simulink model "sschdlexVariableResistorModel"  (R2026a)
settings: Solver=VariableStepAuto  StopTime=.25
libraries: fl_lib x5, nesl_utility x4
settings Model: Creator=The MathWorks, Inc.  LastModifiedBy=The MathWorks, Inc.
settings SimscapeCC: SimscapeNominalValues="[{\"value\":\"1\",\"unit\":\"A\"},{\"value\":\"1\",\"unit\":\"bar\"},{\"value\":\"1\",\"unit\":\"cm^2\"},{\"value\":\"1\",\"unit\":\"cm^3/s\"},{\"value\":\"1\",\"unit\":\"kJ/kg\"},{\"value\":\"1\",\"unit\":\"kW\"},{\"value\":\"1\",\"unit\":\"l\"},{\"value\":\"1\",\"unit\":\"N\"},{\"value\":\"1\",\"unit\":\"N*m\"},{\"value\":\"1\",\"unit\":\"V\"}]"  SimscapeLogType=none  SimscapeLogDataHistory=5000.0

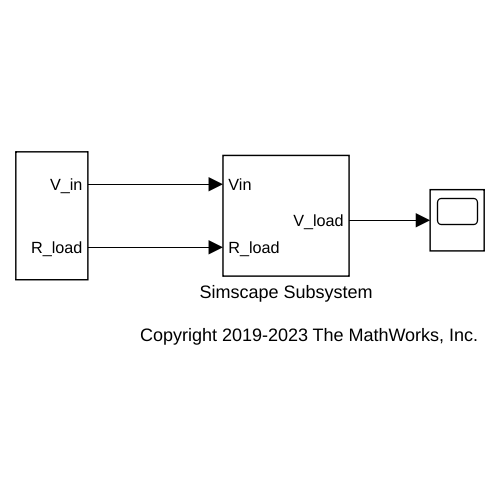
[thumbnail: Simulink's stored preview of the top-level diagram]
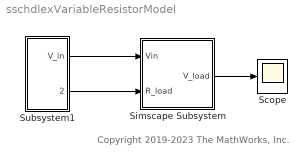
== system sschdlexVariableResistorModel ==
  note: Copyright 2019-2023 The MathWorks, Inc.
  Scope : Scope
      settings: ActiveDisplayYMinimum=-1.68736  ActiveDisplayYMaximum=15.18624
  Simscape Subsystem : Subsystem
  Subsystem1 : Subsystem
  wires:
  Simscape Subsystem/1(V_load) -> Scope/1
  Subsystem1/1(V_in) -> Simscape Subsystem/1(Vin)
  Subsystem1/2(R_load) -> Simscape Subsystem/2(R_load)

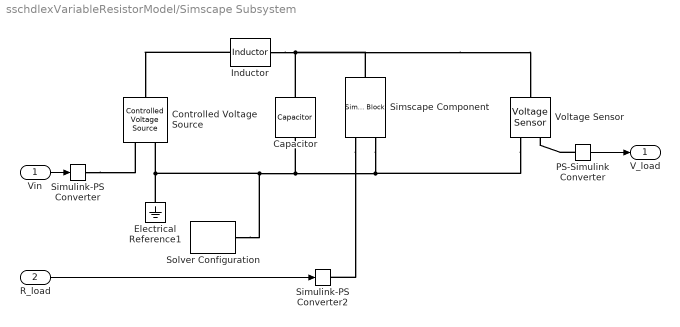
== system sschdlexVariableResistorModel/Simscape Subsystem ==
  Vin : Inport
  R_load : Inport  Port=2
  Capacitor : fl_lib/Electrical/Electrical Elements/Capacitor  c=1e-6 F  r=1e-6 Ohm  g=0 1/Ohm  i_specify=off  i_priority=None  i=0 A  i_nominal_specify=off  i_nominal_value=1  i_nominal_unit=A  v_specify=off  v_priority=None  v=0 V  v_nominal_specify=off  v_nominal_value=1  v_nominal_unit=V  vc_specify=off  vc_priority=High  vc=0 V  vc_nominal_specify=off  vc_nominal_value=1  vc_nominal_unit=V
  Controlled Voltage Source : fl_lib/Electrical/Electrical Sources/Controlled Voltage Source
  Electrical Reference1 : fl_lib/Electrical/Electrical Elements/Electrical Reference
  Inductor : fl_lib/Electrical/Electrical Elements/Inductor  l=1e-3 H  r=0 Ohm  g=1e-9 1/Ohm  i_specify=off  i_priority=None  i=0 A  i_nominal_specify=off  i_nominal_value=1  i_nominal_unit=A  v_specify=off  v_priority=None  v=0 V  v_nominal_specify=off  v_nominal_value=1  v_nominal_unit=V  i_L_specify=off  i_L_priority=High  i_L=0 A  i_L_nominal_specify=off  i_L_nominal_value=1  i_L_nominal_unit=A
  PS-Simulink Converter : nesl_utility/PS-Simulink Converter  PhysicalDomain=network_engine_domain  SubClassName=ps_output  LeftPortType=input  RightPortType=output  PseudoPeriodic=off  Frequencies=[]  VectorFormat=1-D array  Unit=1  AffineConversion=off
  Simscape Component : SimscapeComponentBlock  SourceFile=PiecewiseConstantResistor  ComponentPath=PiecewiseConstantResistor  ComponentVariants="[\"PiecewiseConstantResistor\"]"  ComponentVariantNames="[\"PiecewiseConstantResistor\"]"  ClassName=PiecewiseConstantResistor  SchemaVersion=1  Rmin=1e-6 Ohm  Rtol=1e-6 Ohm  i_specify=off  i_priority=None  i=0 A  i_nominal_specify=off  i_nominal_value=1  i_nominal_unit=A  v_specify=off  v_priority=None  v=0 V  v_nominal_specify=off  v_nominal_value=1  v_nominal_unit=V
      settings: CopyFcn=simscape.sscblock.internal.componentBlockCallback(gcbh,'COPY')  PreCopyFcn=simscape.sscblock.internal.componentBlockCallback(gcbh,'PRECOPY')  PreDeleteFcn=simscape.sscblock.internal.componentBlockCallback(gcbh,'PREDELETE')
      mask Type: Piecewise-Constant Resistor
  Simulink-PS Converter : nesl_utility/Simulink-PS Converter  PhysicalDomain=network_engine_domain  SubClassName=ps_input  LeftPortType=input  RightPortType=output  PseudoPeriodic=off  Frequencies=[]  NoiseDistribution=none  NoiseParameters=[]  Unit=1  AffineConversion=off  FilteringAndDerivatives=provide  SimscapeFilterOrder=1  InputFilterTimeConstant=0.001  UdotUserProvided=0
  Simulink-PS Converter2 : nesl_utility/Simulink-PS Converter  PhysicalDomain=network_engine_domain  SubClassName=ps_input  LeftPortType=input  RightPortType=output  PseudoPeriodic=off  Frequencies=[]  NoiseDistribution=none  NoiseParameters=[]  Unit=1  AffineConversion=off  FilteringAndDerivatives=provide  SimscapeFilterOrder=1  InputFilterTimeConstant=0.001  UdotUserProvided=0
  Solver Configuration : nesl_utility/Solver Configuration  PhysicalDomain=network_engine_domain  SubClassName=solver  LeftPortType=input  RightPortType=generic  Tones=[]  Harmonics=[]  SimulateNoise=off  Profile=off  UseLocalSampling=off  EnableSwitchedLinearOptims=on  FrequencyDomain=off  UseCCode=off  RelTol=0.001  AbsTol=1e-06  MinStep=1e-09  ToWorkspace=off  RevertToSquareIcSolve=off  NumHomotopyIterations=100  PhasorMode=off  PhasorModeNumHarmonics=1  ConsistencySolver=NEWTON_FTOL  CanonicalOrdering=UNORDERED  OptimizeIntermediates=UNOPTIMIZED  IndexReductionMethod=DerivativeReplacement  DoDC=off  ResidualTolerance=1e-09  ConsistencyTolSource=GLOBAL  ConsistencyAbsTol=0.001  ConsistencyRelTol=0.001  ConsistencyTolFactor=0.001  UseLocalSolver=on  LocalSolverChoice=NE_BACKWARD_EULER_ADVANCER  ResolveIndetEquations=on  FunctionEvalNumThread=1  LocalSolverSampleTime=1e-3  DoFixedCost=on  MaxNonlinIter=3  MaxModeIter=2  ComputeImpulses=off  ImpulseIterations=2  LinearAlgebra=auto  LinearAlgebraNumThread=0  EquationFormulation=NE_TIME_EF  DelaysMemoryBudget=1024  AutomaticFiltering=on  FilteringTimeConstant=0.001  PartitionStorageMethod=AS_NEEDED  PartitionMemoryBudget=1024  PartitionMethod=FAST  MultibodyUseLocalSolver=off  MultibodyLocalSolverChoice=ODE1  MultibodyLocalSolverSampleTime=0.001
  Voltage Sensor : fl_lib/Electrical/Electrical Sensors/Voltage Sensor
  V_load : Outport  VectorParamsAs1DForOutWhenUnconnected=off
  wires:
  R_load/1 -> Simulink-PS Converter2/1
  PS-Simulink Converter/1 -> V_load/1
  Vin/1 -> Simulink-PS Converter/1
  connections:
  Inductor/RConn1 -- Simscape Component/RConn1 -- Voltage Sensor/LConn1 -- Capacitor/LConn1
  Solver Configuration/RConn1 -- Controlled Voltage Source/RConn2 -- Electrical Reference1/LConn1 -- Simscape Component/LConn2 -- Voltage Sensor/RConn2 -- Capacitor/RConn1
  Simulink-PS Converter/RConn1 -- Controlled Voltage Source/RConn1
  Inductor/LConn1 -- Controlled Voltage Source/LConn1
  PS-Simulink Converter/LConn1 -- Voltage Sensor/RConn1
  Simscape Component/LConn1 -- Simulink-PS Converter2/RConn1

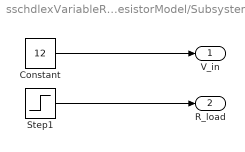
== system sschdlexVariableResistorModel/Subsystem1 ==
  Constant : Constant  Value=12
  Step1 : Step  Time=.1  InitialValue=2  FinalValue=3  SampleTime=1e-3
  V_in : Outport  VectorParamsAs1DForOutWhenUnconnected=off
  R_load : Outport  Port=2  VectorParamsAs1DForOutWhenUnconnected=off
  wires:
  Constant/1 -> V_in/1
  Step1/1 -> R_load/1
